simulink model "fourth_lab"  (R2025b)
settings: Solver=VariableStepAuto  StartTime=0.0  StopTime=10.0  RelTol=1e-3
values from neighbouring files (symbols this model uses):
  vx0 = v0*cos(alpha)    [lab4.m]
  vy0 = v0*sin(alpha)    [lab4.m]
settings Model: Creator=reino  LastModifiedBy=reino

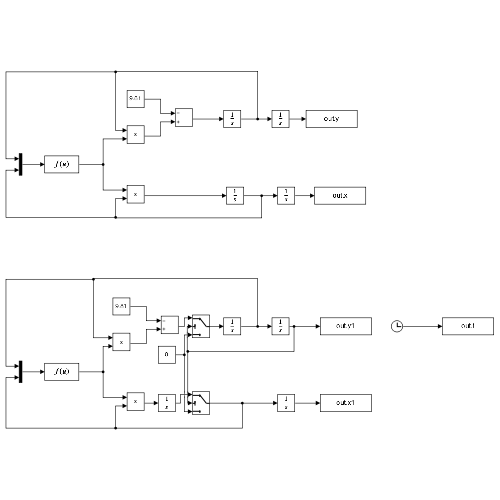
[thumbnail: Simulink's stored preview of the top-level diagram]
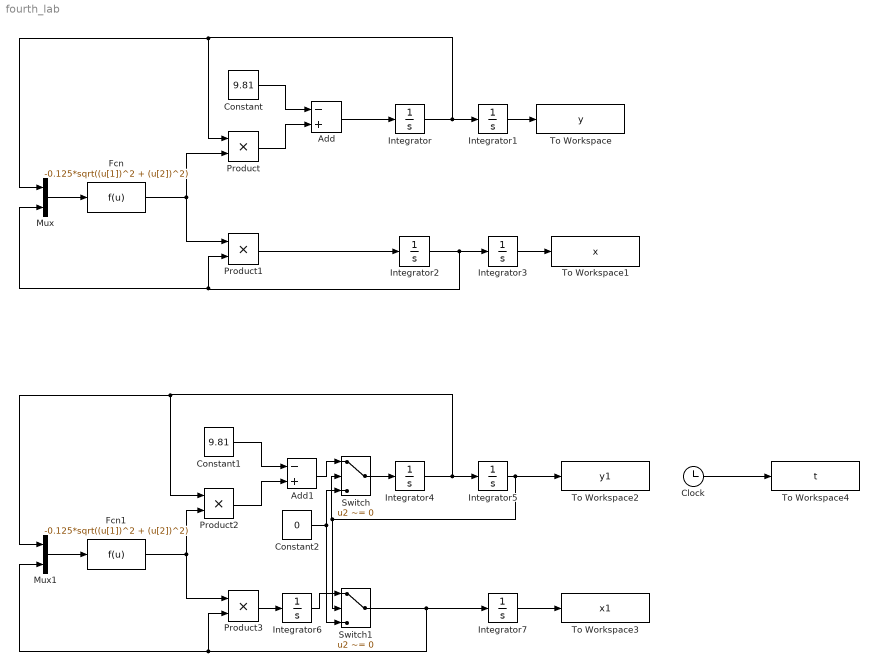
== system fourth_lab ==
  Add : Sum  Inputs=-+
  Add1 : Sum  Inputs=-+
  Clock : Clock
  Constant : Constant  Value=9.81
  Constant1 : Constant  Value=9.81
  Constant2 : Constant  Value=0
  Fcn : Fcn  Expr=-0.125*sqrt((u[1])^2 + (u[2])^2)
  Fcn1 : Fcn  Expr=-0.125*sqrt((u[1])^2 + (u[2])^2)
  Integrator : Integrator  InitialCondition=vy0
  Integrator{1,3,5,7} (4 alike) : Integrator
  Integrator2 : Integrator  InitialCondition=vx0
  Integrator4 : Integrator  InitialCondition=vy0
  Integrator6 : Integrator  InitialCondition=vx0
  Mux : Mux  Inputs=2
  Mux1 : Mux  Inputs=2
  Product{,1..3} (4 alike) : Product
  Switch : Switch  Criteria=u2 ~= 0  SaturateOnIntegerOverflow=off  InputSameDT=off
  Switch1 : Switch  Criteria=u2 ~= 0  SaturateOnIntegerOverflow=off  InputSameDT=off
  To Workspace : ToWorkspace  VariableName=y  SaveFormat=Timeseries  SampleTime=-1
  To Workspace1 : ToWorkspace  VariableName=x  SaveFormat=Timeseries  SampleTime=-1
  To Workspace2 : ToWorkspace  VariableName=y1  SaveFormat=Timeseries  SampleTime=-1
  To Workspace3 : ToWorkspace  VariableName=x1  SaveFormat=Timeseries  SampleTime=-1
  To Workspace4 : ToWorkspace  VariableName=t  SaveFormat=Timeseries  SampleTime=-1
  wires:
  Fcn/1 -> Product/2, Product1/1
  Constant/1 -> Add/1
  Product/1 -> Add/2
  Add/1 -> Integrator/1
  Integrator/1 -> Mux/1, Product/1, Integrator1/1
  Integrator2/1 -> Mux/2, Product1/2, Integrator3/1
  Product1/1 -> Integrator2/1
  Integrator3/1 -> To Workspace1/1
  Integrator1/1 -> To Workspace/1
  Mux/1 -> Fcn/1
  Integrator4/1 -> Mux1/1, Product2/1, Integrator5/1
  Constant1/1 -> Add1/1
  Integrator5/1 -> Switch1/2, Switch/2, To Workspace2/1
  Product2/1 -> Add1/2
  Integrator7/1 -> To Workspace3/1
  Fcn1/1 -> Product2/2, Product3/1
  Mux1/1 -> Fcn1/1
  Add1/1 -> Switch/1
  Switch/1 -> Integrator4/1
  Constant2/1 -> Switch/3, Switch1/3
  Product3/1 -> Integrator6/1
  Integrator6/1 -> Switch1/1
  Switch1/1 -> Mux1/2, Product3/2, Integrator7/1
  Clock/1 -> To Workspace4/1
